simulink model "newest_singleprop"  (R2026b)
settings: Solver=VariableStepAuto  StopTime=60
values from neighbouring files (symbols this model uses):
  data_CP = static_data(:, 5)    [data_manipulation.m]    (also in initialize_propulsion.m)
  data_CT = static_data(:, 4)    [data_manipulation.m]    (also in initialize_propulsion.m)
  g = 9.81    [initialize_propulsion.m]    (also in run_comparisons.mat)
  prop_d = .0254 * prop_inches    (= 0.4318)    [initialize_propulsion.m]    (also in run_comparisons.mat)
  rho_reference = 1.212    [analyze_prop_db.m]    (also in data_manipulation.m; initialize_propulsion.m)
  rho_sim = rho_reference    (= 1.212)    [data_manipulation.m]    (also in initialize_propulsion.m)
libraries: fl_lib x29, nesl_utility x16, sdl_lib x1, batteryecm_lib x1, ee_lib x1
settings Model: Creator=123na  LastModifiedBy=brielle
settings DataIOCC: InspectSignalLogs=on
settings OptimizationCC: BlockReduction=off  BufferReuse=off  DefaultParameterBehavior=Inlined
settings SimscapeCC: SimscapeUseEnergyAccounting=off

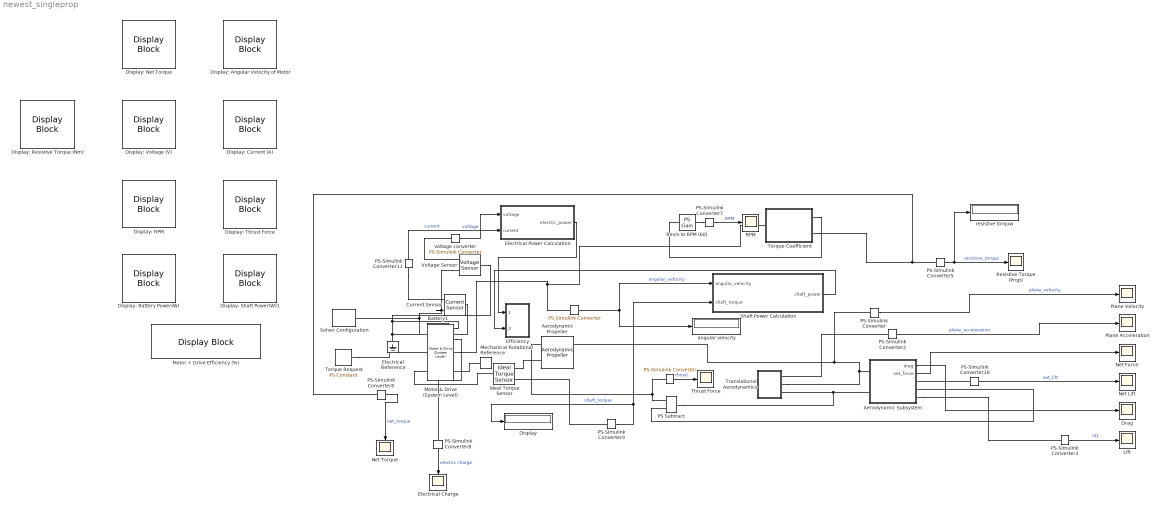
== system newest_singleprop ==
  " " : nesl_utility/PS-Simulink Converter  PhysicalDomain=network_engine_domain  SubClassName=ps_output  LeftPortType=input  RightPortType=output  PseudoPeriodic=off  Frequencies=[]  VectorFormat=inherit  Unit=N  AffineConversion=off
  "  " : nesl_utility/PS-Simulink Converter  PhysicalDomain=network_engine_domain  SubClassName=ps_output  LeftPortType=input  RightPortType=output  PseudoPeriodic=off  Frequencies=[]  VectorFormat=inherit  Unit=inherit  AffineConversion=off
  " Rev/s to RPM (60)" : fl_lib/Physical Signals/Functions/PS Gain  gain=60
  Aerodynamic Propeller : sdl_lib/Engines & Motors/Aerodynamic Propeller  parameterization=sdl.enum.AerodynamicPropellerParameterization.Constant  enable_collective_pitch_control=false  enable_transverse_flow=false  direction=sdl.enum.PropellerDirection.Positive  root_pitch=0 deg  D=prop_d m  kt_const=data_CT(4)  kp_const=data_CP(4)  kt_poly_fixed=[.002, .0006, -.0509, .0617]  kp_poly_fixed=[-.0752, .0577, -.0622, .16]  pitch_angle_TLU=[-15, 15, 25, 35, 45] deg  kt_poly_TLU=[.0002, -.00041, -.036, .03; .00026, -.00056, -.048, .04; .002, .00063, -.051, .062; .0014, -.0016, -.048, .087; .00087, -.0036, -.041, .12]  kp_poly_TLU=[-.1, .031, .0055, .088; -.081, -.025, .0044, .07; -.075, .058, -.062, .16; -.052, .065, -.08, .3; -.031, .057, -.069, .4]  J_TLU=[.01, .3, .625, 1.55, 2, 2.6]  kt_TLU_1D=[.0614, .0473, .0318, -.0127, -.0343, -.063]  kp_TLU_1D=[.1496, .1314, .116, -.0521, -.1503, -.2813]  kt_TLU_2D=[.00019, .013, .0048, -.017, -.03, -.045; .00039, .025, .0096, -.037, -.06, -.09; .00061, .047, .032, -.013, -.034, -.063; .00086, .072, .057, .014, -.0076, -.036; .12, .104, .09, .049, .029, .0019]  kp_TLU_2D=[.029, .029, .016, .06, .009, -.16; .059, .054, .031, -.12, -.19, -.29; .15, .13, .12, -.052, -.15, -.28; .26, .24, .22, .097, -.04, -.25; .39, .39, .38, .32, .24, .062]  beta_TLU=linspace(0, 360, 10) deg  Ct_TLU_1D=0.035 * sind(linspace(0, 360, 10) - 200)  Cq_TLU_1D=0.010 * sind(linspace(0, 360, 10) - 200)  Ct_TLU_2D=[0.01 * sind(linspace(0, 360, 10) - 200); 0.020 * sind(linspace(0, 360, 10) - 200); 0.035 * sind(linspace(0, 360, 10) - 200); 0.04 * sind(linspace(0, 360, 10) - 200); 0.06 * sind(linspace(0, 360, 10) - 200)]  Cq_TLU_2D=[0.0005 * sind(linspace(0, 360, 10) - 200); 0.0015 * sind(linspace(0, 360, 10) - 200); 0.0025 * sind(linspace(0, 360, 10) - 200); 0.0035 * sind(linspace(0, 360, 10) - 200); 0.0045 * sind(linspace(0, 360, 10) - 200)]  n_blades=2  radial_TLU=[.1, .12, .2, .4, .6, .8, 1]  twist_TLU=[30, 35, 50, 30, 20, 15, 10] deg  chord_TLU=[.0676, .0666, .0824, .1025, .0885, .0598, .0133]  alpha_TLU=-180 : 10 : 180 deg  Cl_TLU=[.1326, .1326, .1274, .1274, .1274, .1274, .1274; .3626, .3626, .5002, .5002, .5002, .5002, .5002; .5528, .5528, .8007, .8007, .8007, .8007, .8007; .7256, .7256, 1.0125, 1.0125, 1.0125, 1.0125, 1.0125; .8016, .8016, 1.1556, 1.1556, 1.1556, 1.1556, 1.1556; .7873, .7873, 1.1604, 1.1604, 1.1604, 1.1604, 1.1604; .7031, .7031, 1.0493, 1.0493, 1.0493, 1.0493, 1.0493; .5423, .5423, .7973, .7973, .7973, .7973, .7973; .3537, .3537, .4332, .4332, .4332, .4332, .4332; .1155, .1155, -.0376, -.0376, -.0376, -.0376, -.0376; -.1045, -.1045, -.4096, -.4096, -.4096, -.4096, -.4096; -.2999, -.2999, -.672, -.672, -.672, -.672, -.672; -.4401, -.4401, -.9343, -.9343, -.9343, -.9343, -.9343; -.5186, -.5186, -1.0477, -1.0477, -1.0477, -1.0477, -1.0477; -.5303, -.5303, -1.0387, -1.0387, -1.0387, -1.0387, -1.0387; -.5073, -.5073, -.9565, -.9565, -.9565, -.9565, -.9565; -.442, -.442, -.7713, -.7713, -.7713, -.7713, -.7713; -.2658, -.2658, -.4832, -.4832, -.4832, -.4832, -.4832; .4109, .4109, .3629, .3629, .3629, .3629, .3629; 1.1635, 1.1635, 1.3779, 1.3779, 1.3779, 1.3779, 1.3779; 1.2412, 1.2412, 1.4033, 1.4033, 1.4033, 1.4033, 1.4033; .7434, .7434, 1.3453, 1.3453, 1.3453, 1.3453, 1.3453; .7908, .7908, 1.2862, 1.2862, 1.2862, 1.2862, 1.2862; .7525, .7525, 1.1562, 1.1562, 1.1562, 1.1562, 1.1562; .6722, .6722, .9487, .9487, .9487, .9487, .9487; .5324, .5324, .7047, .7047, .7047, .7047, .7047; .3365, .3365, .382, .382, .382, .382, .382; .0529, .0529, -.0229, -.0229, -.0229, -.0229, -.0229; -.2728, -.2728, -.316, -.316, -.316, -.316, -.316; -.4135, -.4135, -.6195, -.6195, -.6195, -.6195, -.6195; -.5087, -.5087, -.7847, -.7847, -.7847, -.7847, -.7847; -.5342, -.5342, -.8419, -.8419, -.8419, -.8419, -.8419; -.5166, -.5166, -.7658, -.7658, -.7658, -.7658, -.7658; -.4321, -.4321, -.5707, -.5707, -.5707, -.5707, -.5707; -.2864, -.2864, -.3098, -.3098, -.3098, -.3098, -.3098; -.1073, -.1073, -.0893, -.0893, -.0893, -.0893, -.0893; .1326, .1326, .1274, .1274, .1274, .1274, .1274]  Cd_TLU=[.0055, .0055, .3904, .3904, .3904, .3904, .3904; .0774, .0774, .449, .449, .449, .449, .449; .2412, .2412, .5915, .5915, .5915, .5915, .5915; .4342, .4342, .8307, .8307, .8307, .8307, .8307; .679, .679, 1.0909, 1.0909, 1.0909, 1.0909, 1.0909; .9003, .9003, 1.3868, 1.3868, 1.3868, 1.3868, 1.3868; 1.0825, 1.0825, 1.6565, 1.6565, 1.6565, 1.6565, 1.6565; 1.2281, 1.2281, 1.875, 1.875, 1.875, 1.875, 1.875; 1.3205, 1.3205, 2.017, 2.017, 2.017, 2.017, 2.017; 1.3234, 1.3234, 2.0407, 2.0407, 2.0407, 2.0407, 2.0407; 1.2391, 1.2391, 1.9513, 1.9513, 1.9513, 1.9513, 1.9513; 1.0963, 1.0963, 1.7643, 1.7643, 1.7643, 1.7643, 1.7643; .8978, .8978, 1.5048, 1.5048, 1.5048, 1.5048, 1.5048; .6525, .6525, 1.2281, 1.2281, 1.2281, 1.2281, 1.2281; .4203, .4203, .838, .838, .838, .838, .838; .2428, .2428, .5434, .5434, .5434, .5434, .5434; .0951, .0951, .2517, .2517, .2517, .2517, .2517; .0292, .0292, .0698, .0698, .0698, .0698, .0698; .0148, .0148, .0267, .0267, .0267, .0267, .0267; .0808, .0808, .0509, .0509, .0509, .0509, .0509; .2429, .2429, .1561, .1561, .1561, .1561, .1561; .5019, .5019, .3927, .3927, .3927, .3927, .3927; .7217, .7217, .7438, .7438, .7438, .7438, .7438; .9336, .9336, 1.1277, 1.1277, 1.1277, 1.1277, 1.1277; 1.0984, 1.0984, 1.4838, 1.4838, 1.4838, 1.4838, 1.4838; 1.2274, 1.2274, 1.7877, 1.7877, 1.7877, 1.7877, 1.7877; 1.3016, 1.3016, 1.9779, 1.9779, 1.9779, 1.9779, 1.9779; 1.3305, 1.3305, 2.0516, 2.0516, 2.0516, 2.0516, 2.0516; 1.2889, 1.2889, 1.9974, 1.9974, 1.9974, 1.9974, 1.9974; 1.1677, 1.1677, 1.8463, 1.8463, 1.8463, 1.8463, 1.8463; 1.0076, 1.0076, 1.5699, 1.5699, 1.5699, 1.5699, 1.5699; .8068, .8068, 1.2596, 1.2596, 1.2596, 1.2596, 1.2596; .5688, .5688, .9493, .9493, .9493, .9493, .9493; .3604, .3604, .6154, .6154, .6154, .6154, .6154; .1802, .1802, .5015, .5015, .5015, .5015, .5015; .0699, .0699, .4265, .4265, .4265, .4265, .4265; .0055, .0055, .3904, .3904, .3904, .3904, .3904]  interp_method=simscape.enum.interpolation.linear  extrap_method=simscape.enum.extrapolation.linear  n_blade_discretization=10  n_azimuthal_discretization=10  density_spec=foundation.enum.constant_variable.constant  rho=rho_reference kg/m^3  rotational_ports=sdl.enum.ConnectionType.Conserving  translational_ports=sdl.enum.ConnectionType.PS  model_inertia=true  propeller_inertia=0.00001 kg*m^2  propeller_mass=10 kg  efficiency_sensor=false  n_thr=0.001 Hz  k_thr=0.001  P_thr=0.01 W  operation_check=simscape.enum.assert.action.warn  expose_port_C=false  w_specify=on  w_priority=High  w=0 rad/s  w_nominal_specify=off  w_nominal_value=1  w_nominal_unit=rad/s  Q_specify=off  Q_priority=None  Q=0 N*m  Q_nominal_specify=off  Q_nominal_value=1  Q_nominal_unit=N*m  v_specify=off  v_priority=None  v=0 m/s  v_nominal_specify=off  v_nominal_value=1  v_nominal_unit=m/s  thrust_specify=off  thrust_priority=None  thrust=0 N  thrust_nominal_specify=off  thrust_nominal_value=1  thrust_nominal_unit=N
  Aerodynamic Subsystem : Subsystem
  Battery1 : batteryecm_lib/Battery  Vnom=22.2 V  prm_dir=simscape.enum.battery.prm_dir.disabled  R1_dis=2 Ohm  R1_ch=2 Ohm  R1=15 mOhm  prm_AH=simscape.enum.battery.prm_AH.finite  AH=4 A*hr  V1=21.3 V  AH1=0.48 Ah  prm_R2=simscape.enum.battery.prm_R2.disabled  R2=2000 Ohm  Tmeas=298.15 K  charge_measurement_port=simscape.enum.battery.enable.yes  prm_dyn=simscape.enum.battery.prm_dyn.off  Rp1=0.005 Ohm  tau1=30 s  Rp2=0.005 Ohm  tau2=30 s  Rp3=0.005 Ohm  tau3=30 s  Rp4=0.005 Ohm  tau4=30 s  Rp5=0.005 Ohm  tau5=30 s  prm_fade=simscape.enum.battery.prm_fade.disabled  N_fade=100  AH_fade=45 A*hr  R1_fade=2.02 Ohm  R1_ch_fade=2.02 Ohm  V1_fade=10.35 V  prm_age=simscape.enum.battery.prm_age.disabled  prm_age_OCV=simscape.enum.battery.prm_age_OCV.OCV  OCV_age=0.9  SOC_age=60  Tmeas_age=298.15 K  delta_time_age_vec=[0] d  temperature_age_vec=[273] K  OCV_scaling_age=2.2134e6  OCV_offset_age=1.632e6  temp_exp_age=0.515833569 V  t_exp_age=0.75  Vnom_T2=12 V  R1_T2=2.2 Ohm  R1_T2_dis=2.2 Ohm  R1_T2_ch=2.2 Ohm  V1_T2=11.4 V  R2_T2=2200 Ohm  Rp1_T2=0.005 Ohm  tau1_T2=30 s  Rp2_T2=0.005 Ohm  tau2_T2=30 s  Rp3_T2=0.005 Ohm  tau3_T2=30 s  Rp4_T2=0.005 Ohm  tau4_T2=30 s  Rp5_T2=0.005 Ohm  tau5_T2=30 s  Tmeas2=273.15 K  thermal_port=simscape.enum.thermaleffects.omit  thermal_mass=30000 J/K  i_specify=off  i_priority=None  i=0 A  i_nominal_specify=off  i_nominal_value=1  i_nominal_unit=A  v_specify=off  v_priority=None  v=0 V  v_nominal_specify=off  v_nominal_value=1  v_nominal_unit=V  charge_specify=off  charge_priority=High  charge=50 A*hr  charge_nominal_specify=off  charge_nominal_value=1  charge_nominal_unit=A*hr  num_cycles_specify=off  num_cycles_priority=High  num_cycles=0  num_cycles_nominal_specify=off  num_cycles_nominal_value=1  num_cycles_nominal_unit=1  temperature_specify=off  temperature_priority=High  temperature=298.15 K  temperature_nominal_specify=off  temperature_nominal_value=1  temperature_nominal_unit=K
      settings: LibrarySourceBlock=batt_lib/Cells/Battery
  Current Sensor : fl_lib/Electrical/Electrical Sensors/Current Sensor
  Display : Display
  Display: Angular Velocity of Motor : DisplayBlock  LabelPosition=Hide  Transparency=1  GridColor=[0.502, 0.502, 0.502]
  Display: Battery Power(W) : DisplayBlock  LabelPosition=Hide  Format=Integer  Transparency=1  GridColor=[0.0, 0.0, 1.0]
  Display: Current (A) : DisplayBlock  LabelPosition=Hide  Transparency=1  GridColor=[0.502, 0.502, 0.502]
  Display: Net Torque : DisplayBlock  LabelPosition=Hide  Transparency=1  GridColor=[0.502, 0.502, 0.502]
  Display: RPM : DisplayBlock  LabelPosition=Hide  Format=Integer  Transparency=1  GridColor=[0.0, 0.0, 1.0]
  Display: Resistive Torque (Nm) : DisplayBlock  LabelPosition=Hide  Transparency=1  GridColor=[0.502, 0.502, 0.502]
  Display: Shaft Power(W)1 : DisplayBlock  LabelPosition=Hide  Transparency=1  GridColor=[0.0, 0.0, 1.0]
  Display: Thrust Force : DisplayBlock  LabelPosition=Hide  Transparency=1  GridColor=[0.502, 0.502, 0.502]
  Display: Voltage (V) : DisplayBlock  LabelPosition=Hide  Transparency=1  GridColor=[0.502, 0.502, 0.502]
  Drag : Scope
      settings: ActiveDisplayYMinimum=-14.344967530290399  ActiveDisplayYMaximum=129.10470777261361  DataLoggingVariableName=ScopeData8
  Efficiency : Subsystem
  Electrical Charge : Scope
      settings: ActiveDisplayYMinimum=160492.22040625822  ActiveDisplayYMaximum=182167.5310659713  DataLoggingVariableName=ScopeData10
  Electrical Power Calculation : Subsystem
  Electrical Reference : fl_lib/Electrical/Electrical Elements/Electrical Reference
  Ideal Torque Sensor : fl_lib/Mechanical/Mechanical Sensors/Ideal Torque Sensor
  Lift : Scope
      settings: ActiveDisplayYMinimum=-49.526573340247545  ActiveDisplayYMaximum=445.73916006222805  DataLoggingVariableName=ScopeData7
  Mechanical Rotational Reference : fl_lib/Mechanical/Rotational Elements/Mechanical Rotational Reference
  Motor & Drive (System Level) : ee_lib/Electromechanical/Motor & Drive (System Level)  torque_speed_param=ee.enum.electromech.envelope.torque_power  overtorque_param=ee.enum.electromech.overtorque.no  T_t=[.09, .08, .07, 0] N*m  T_t_intermittent=[.36, .32, .28, 0] N*m  T_t_2D=[.09, .09, .09; .08, .08, .08; .07, .07, .07; 0, 0, 0] N*m  T_t_intermittent_2D=[.36, .36, .36; .32, .32, .32; .28, .28, .28; 0, 0, 0] N*m  w_t=[0, 3750, 7500, 8000] rpm  vdc_t=[6, 12, 24] V  torque_max=5.5 N*m  power_max=900 W  torque_max_intermittent=0.4 N*m  power_max_intermittent=120 W  time_overtorque=30 s  time_recover=60 s  Tc=0.02 s  EnableSwitch=false  losses_param=1  eff=88  w_eff=6000 rpm  T_eff=4 N*m  Piron=0 W  Pbase=0 W  w_eff_vec=[-8000, -4000, 0, 4000, 8000] rpm  T_eff_vec=[0, .03, .06, .09] N*m  v_eff_vec=[100, 250, 400] V  losses_mat=[1.49, 1.67, 2.21, 3.1; .42, .69, 1.14, 2.03; .06, .24, .78, 1.68; .42, .69, 1.14, 2.03; 1.49, 1.67, 2.21, 3.1] W  efficiency_mat=[95, 95, 95, 95; 95, 95, 95, 95; 95, 95, 95, 95; 95, 95, 95, 95; 95, 95, 95, 95]  losses_mat_3D=ones(5, 4, 3) W  efficiency_mat_3D=95 * ones(5, 4, 3)  Res=0.016 Ohm  J=5e-6 kg*m^2  lam=1e-5 N*m*s/rad  speed0=0 rpm  faulted_specify=off  faulted_priority=None  faulted=0  faulted_nominal_specify=off  faulted_nominal_value=1  faulted_nominal_unit=1  isSwitchedOff_specify=off  isSwitchedOff_priority=None  isSwitchedOff=0  isSwitchedOff_nominal_specify=off  isSwitchedOff_nominal_value=1  isSwitchedOff_nominal_unit=1  torqueLimitContinuous_specify=off  torqueLimitContinuous_priority=None  torqueLimitContinuous=0 N*m  torqueLimitContinuous_nominal_specify=off  torqueLimitContinuous_nominal_value=1  torqueLimitContinuous_nominal_unit=N*m  TabulateLossesForMultipleTemperatures=false  alpha=3.93e-3 1/K  Tmeas=25 degC  TmeasVec=[25, 75, 125] degC  Tmeas2=125 degC  losses_mat_T2=[1.49, 1.74, 2.49, 3.74; .42, .67, 1.42, 2.67; .06, .31, 1.06, 2.31; .42, .67, 1.42, 2.67; 1.49, 1.74, 2.49, 3.74] W  efficiency_mat_T2=[95, 95, 95, 95; 95, 95, 95, 95; 95, 95, 95, 95; 95, 95, 95, 95; 95, 95, 95, 95]  losses_mat_3D_T2=ones(5, 4, 3) W  efficiency_mat_3D_T2=95 * ones(5, 4, 3)  lossesMatMultipleTemperatures=ones(5, 4, 3) W  efficiencyMatMultipleTemperatures=95 * ones(5, 4, 3)  lossesMat4DMultipleTemperatures=ones(5, 4, 3, 3) W  efficiencyMat4DMultipleTemperatures=95 * ones(5, 4, 3, 3)  thermal_mass=100 J/K  initial_temperature=25 degC
  Motor + Drive Efficiency (%) : DisplayBlock  LabelPosition=Hide  Transparency=1  GridColor=[0.0, 0.0, 1.0]
  Net Force : Scope
      settings: ActiveDisplayYMinimum=-4.5427625845531994  ActiveDisplayYMaximum=40.884863260978804  DataLoggingVariableName=ScopeData5
  Net Lift : Scope
      settings: ActiveDisplayYMinimum=-156.32019566352511  ActiveDisplayYMaximum=338.9455409717259  DataLoggingVariableName=ScopeData12
  Net Torque : Scope
      settings: ActiveDisplayYMinimum=2.5365925575733379  ActiveDisplayYMaximum=5.2737119380474073  DataLoggingVariableName=ScopeData4
  PS Subtract : fl_lib/Physical Signals/Functions/PS Subtract
  PS-Simulink Converter{,2..3,5..10} (9 alike) : nesl_utility/PS-Simulink Converter  PhysicalDomain=network_engine_domain  SubClassName=ps_output  LeftPortType=input  RightPortType=output  PseudoPeriodic=off  Frequencies=[]  VectorFormat=inherit  Unit=inherit  AffineConversion=off
  PS-Simulink Converter11 : nesl_utility/PS-Simulink Converter  PhysicalDomain=network_engine_domain  SubClassName=ps_output  LeftPortType=input  RightPortType=output  PseudoPeriodic=off  Frequencies=[]  VectorFormat=inherit  Unit=A  AffineConversion=off
  Plane Acceleration : Scope
      settings: ActiveDisplayYMinimum=-0.565213030160767  ActiveDisplayYMaximum=5.0869172714469038
  Plane Velocity : Scope
      settings: ActiveDisplayYMinimum=-4.7776171506476794  ActiveDisplayYMaximum=42.998554355829121  DataLoggingVariableName=ScopeData6
  RPM : Scope
      settings: ActiveDisplayYMinimum=-379.69821594020021  ActiveDisplayYMaximum=3417.2839434618027  DataLoggingVariableName=ScopeData9
  Resistive Torque (Prop) : Scope
      settings: ActiveDisplayYMinimum=-0.15553318378531714  ActiveDisplayYMaximum=1.3997986540678544  DataLoggingVariableName=ScopeData3
  Shaft Power Calculation : Subsystem
  Solver Configuration : nesl_utility/Solver Configuration  PhysicalDomain=network_engine_domain  SubClassName=solver  LeftPortType=input  RightPortType=generic  Tones=[]  Harmonics=[]  SimulateNoise=off  Profile=off  UseLocalSampling=off  EnableSwitchedLinearOptims=on  FrequencyDomain=off  UseCCode=off  RelTol=0.001  AbsTol=0.001  MinStep=1e-09  ToWorkspace=off  RevertToSquareIcSolve=off  NumHomotopyIterations=100  PhasorMode=off  PhasorModeNumHarmonics=1  ConsistencySolver=NEWTON_XTOL_AFTER_FTOL  CanonicalOrdering=UNORDERED  OptimizeIntermediates=UNOPTIMIZED  MulticoreSolverChoice=BACKWARD_EULER  IndexReductionMethod=DerivativeReplacement  DoDC=off  ResidualTolerance=1e-09  ConsistencyTolSource=GLOBAL  ConsistencyAbsTol=0.001  ConsistencyRelTol=0.001  ConsistencyTolFactor=0.001  UseLocalSolver=off  LocalSolverChoice=NE_BACKWARD_EULER_ADVANCER  ResolveIndetEquations=on  FunctionEvalNumThread=1  LocalSolverSampleTime=0.001  DoFixedCost=off  MaxNonlinIter=3  MaxModeIter=2  ComputeImpulses=off  ImpulseIterations=2  LinearAlgebra=auto  LinearAlgebraNumThread=0  EquationFormulation=NE_TIME_EF  DelaysMemoryBudget=1024  AutomaticFiltering=on  FilteringTimeConstant=0.001  PartitionStorageMethod=AS_NEEDED  PartitionMemoryBudget=1024  PartitionMethod=BALANCED  MultibodyUseLocalSolver=off  MultibodyLocalSolverChoice=ODE1  MultibodyLocalSolverSampleTime=0.001
  "Thrust Force " : Scope
      settings: ActiveDisplayYMinimum=-7.0175807682346578  ActiveDisplayYMaximum=63.158226914111935
  Torque Coefficient : Subsystem
  Torque Request : fl_lib/Physical Signals/Sources/PS Constant  constant=2.15 N*m
  Translational Aerodynamics : Subsystem
  Voltage Sensor : fl_lib/Electrical/Electrical Sensors/Voltage Sensor
  angular velocity : Display
  resistive torquw : Display
  voltage converter : nesl_utility/PS-Simulink Converter  PhysicalDomain=network_engine_domain  SubClassName=ps_output  LeftPortType=input  RightPortType=output  PseudoPeriodic=off  Frequencies=[]  VectorFormat=inherit  Unit=inherit  AffineConversion=off
  wires:
  " "/1 -> "Thrust Force "/1  "thrust"
  PS-Simulink Converter/1 -> Plane Velocity/1  "plane_velocity"
  PS-Simulink Converter2/1 -> Plane Acceleration/1  "plane_acceleration"
  PS-Simulink Converter3/1 -> Lift/1  "lift"
  PS-Simulink Converter6/1 -> Net Torque/1  "net_torque"
  PS-Simulink Converter5/1 -> resistive torquw/1, Resistive Torque (Prop)/1  "resistive_torque"
  PS-Simulink Converter7/1 -> RPM/1  "RPM"
  PS-Simulink Converter8/1 -> Electrical Charge/1  "electric charge"
  PS-Simulink Converter10/1 -> Net Lift/1  "net_lift"
  "  "/1 -> Shaft Power Calculation/1(angular_velocity), angular velocity/1  "angular_velocity"
  voltage converter/1 -> Electrical Power Calculation/1(voltage)  "voltage"
  PS-Simulink Converter11/1 -> Electrical Power Calculation/2(current)  "current"
  Electrical Power Calculation/1(electric_power) -> Efficiency/1(electrical power)
  Aerodynamic Subsystem/1(drag) -> Drag/1
  Aerodynamic Subsystem/2(net_force) -> Net Force/1
  PS-Simulink Converter9/1 -> Display/1, Shaft Power Calculation/2(shaft_torque)  "shaft_torque"
  Shaft Power Calculation/1(shaft_power) -> Efficiency/2(shaft power)
  connections:
  Motor & Drive (System Level)/LConn1 -- Voltage Sensor/LConn1 -- Battery1/LConn1 -- Electrical Reference/LConn1
  Voltage Sensor/RConn2 -- Current Sensor/RConn2 -- Battery1/RConn1 -- Solver Configuration/RConn1
  Motor & Drive (System Level)/RConn3 -- Mechanical Rotational Reference/LConn1
  Motor & Drive (System Level)/RConn2 -- Torque Coefficient/LConn1 -- "  "/LConn1
  " "/LConn1 -- Aerodynamic Propeller/LConn1 -- PS Subtract/LConn1
  Torque Request/RConn1 -- Motor & Drive (System Level)/LConn2
  Torque Coefficient/RConn2 -- PS-Simulink Converter6/LConn1 -- PS-Simulink Converter5/LConn1
  " Rev/s to RPM (60)"/RConn1 -- PS-Simulink Converter7/LConn1
  Battery1/LConn2 -- PS-Simulink Converter8/LConn1
  Voltage Sensor/RConn1 -- voltage converter/LConn1
  Motor & Drive (System Level)/RConn1 -- Current Sensor/LConn1
  PS-Simulink Converter11/LConn1 -- Current Sensor/RConn1
  PS-Simulink Converter9/LConn1 -- Ideal Torque Sensor/RConn2
  Ideal Torque Sensor/RConn1 -- Aerodynamic Propeller/LConn2
  Motor & Drive (System Level)/LConn3 -- Ideal Torque Sensor/LConn1
  Torque Coefficient/RConn1 -- " Rev/s to RPM (60)"/LConn1
  PS-Simulink Converter2/LConn1 -- Translational Aerodynamics/RConn1
  Translational Aerodynamics/RConn2 -- PS-Simulink Converter/LConn1 -- Aerodynamic Propeller/RConn1 -- Aerodynamic Subsystem/LConn1
  Translational Aerodynamics/RConn3 -- PS Subtract/RConn1 -- Aerodynamic Subsystem/LConn2
  PS-Simulink Converter10/LConn1 -- Aerodynamic Subsystem/RConn1
  PS Subtract/LConn2 -- Aerodynamic Subsystem/RConn2
  Aerodynamic Subsystem/RConn3 -- PS-Simulink Converter3/LConn1

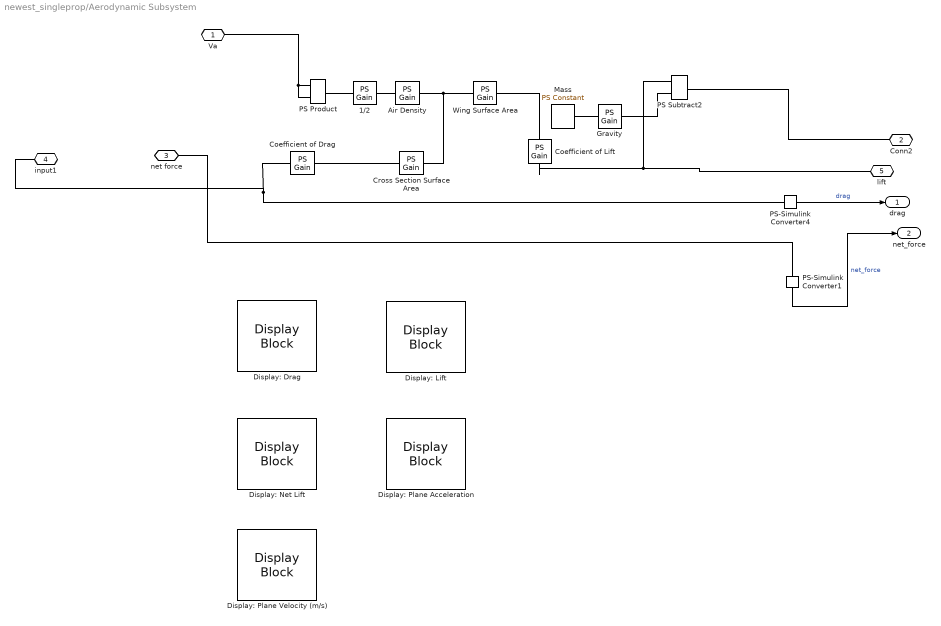
== system newest_singleprop/Aerodynamic Subsystem ==
  1/2 : fl_lib/Physical Signals/Functions/PS Gain  gain=.5
  Air Density : fl_lib/Physical Signals/Functions/PS Gain  gain=rho_sim kg/m^3
  Coefficient of Drag : fl_lib/Physical Signals/Functions/PS Gain  gain=0.06
  Coefficient of Lift : fl_lib/Physical Signals/Functions/PS Gain  gain=.58
  Cross Section Surface Area : fl_lib/Physical Signals/Functions/PS Gain  gain=1.0448384 m^2
  Display: Drag : DisplayBlock  LabelPosition=Hide  Transparency=1  GridColor=[0.502, 0.502, 0.502]
  Display: Lift : DisplayBlock  LabelPosition=Hide  Transparency=1  GridColor=[0.502, 0.502, 0.502]
  Display: Net Lift : DisplayBlock  LabelPosition=Hide  Transparency=1  GridColor=[0.502, 0.502, 0.502]
  Display: Plane Acceleration : DisplayBlock  LabelPosition=Hide  Transparency=1  GridColor=[0.502, 0.502, 0.502]
  Display: Plane Velocity (m/s) : DisplayBlock  LabelPosition=Hide  Transparency=1  GridColor=[0.502, 0.502, 0.502]
  Gravity : fl_lib/Physical Signals/Functions/PS Gain  gain=g m/(s^2)
  Mass : fl_lib/Physical Signals/Sources/PS Constant  constant=mass kg
  PS Product : fl_lib/Physical Signals/Functions/PS Product
  PS Subtract2 : fl_lib/Physical Signals/Functions/PS Subtract
  PS-Simulink Converter1 : nesl_utility/PS-Simulink Converter  PhysicalDomain=network_engine_domain  SubClassName=ps_output  LeftPortType=input  RightPortType=output  PseudoPeriodic=off  Frequencies=[]  VectorFormat=inherit  Unit=inherit  AffineConversion=off
  PS-Simulink Converter4 : nesl_utility/PS-Simulink Converter  PhysicalDomain=network_engine_domain  SubClassName=ps_output  LeftPortType=input  RightPortType=output  PseudoPeriodic=off  Frequencies=[]  VectorFormat=inherit  Unit=inherit  AffineConversion=off
  Wing Surface Area : fl_lib/Physical Signals/Functions/PS Gain  gain=0.87 m^2
  Va : PMIOPort  Side=Left
  Conn2 : PMIOPort  Port=2  Side=Right
  net force : PMIOPort  Port=3  Side=Left
  input1 : PMIOPort  Port=4  Side=Right
  lift : PMIOPort  Port=5  Side=Right
  drag : Outport
  net_force : Outport  Port=2
  wires:
  PS-Simulink Converter1/1 -> net_force/1  "net_force"
  PS-Simulink Converter4/1 -> drag/1  "drag"
  connections:
  Conn2/RConn1 -- PS Subtract2/RConn1
  Coefficient of Lift/LConn1 -- Wing Surface Area/RConn1
  Wing Surface Area/LConn1 -- Cross Section Surface Area/LConn1 -- Air Density/RConn1
  PS Product/RConn1 -- 1/2/LConn1
  Air Density/LConn1 -- 1/2/RConn1
  Gravity/RConn1 -- PS Subtract2/LConn2
  Gravity/LConn1 -- Mass/RConn1
  PS Product/LConn1 -- PS Product/LConn2 -- Va/RConn1
  PS-Simulink Converter1/LConn1 -- net force/RConn1
  Cross Section Surface Area/RConn1 -- Coefficient of Drag/LConn1
  Coefficient of Drag/RConn1 -- input1/RConn1 -- PS-Simulink Converter4/LConn1
  Coefficient of Lift/RConn1 -- PS Subtract2/LConn1 -- lift/RConn1

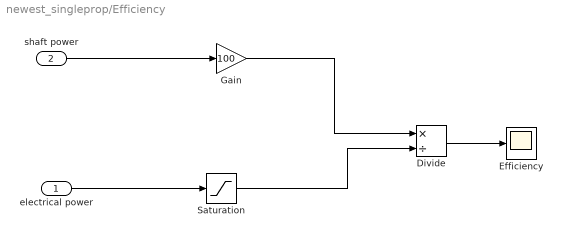
== system newest_singleprop/Efficiency ==
  electrical power : Inport
  shaft power : Inport  Port=2
  Divide : Product  Inputs=*/
  Efficiency : Scope
      settings: ActiveDisplayYMinimum=-54.765164223208942  ActiveDisplayYMaximum=492.8864780088806  DataLoggingVariableName=ScopeData14
  Gain : Gain  Gain=100
  Saturation : Saturate  UpperLimit=inf  LowerLimit=.0001
  wires:
  shaft power/1 -> Gain/1
  electrical power/1 -> Saturation/1
  Divide/1 -> Efficiency/1
  Saturation/1 -> Divide/2
  Gain/1 -> Divide/1

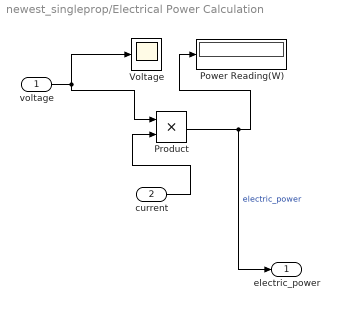
== system newest_singleprop/Electrical Power Calculation ==
  voltage : Inport
  current : Inport  Port=2
  Power Reading(W) : Display
  Product : Product
  Voltage : Scope
      settings: ActiveDisplayYMinimum=21.504198233190788  ActiveDisplayYMaximum=22.408763563943079  DataLoggingVariableName=ScopeData11
  electric_power : Outport
  wires:
  current/1 -> Product/2
  Product/1 -> electric_power/1, Power Reading(W)/1  "electric_power"
  voltage/1 -> Product/1, Voltage/1

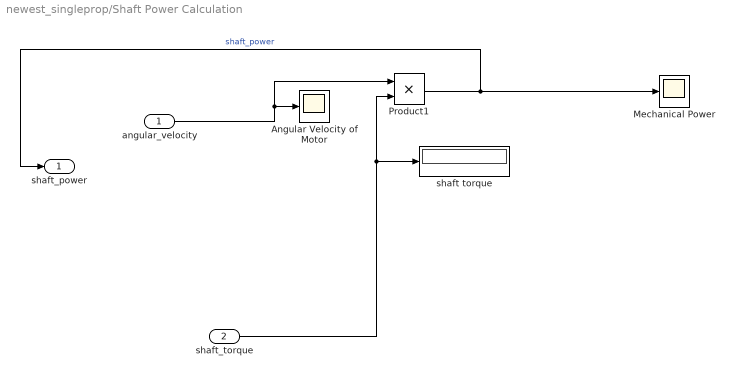
== system newest_singleprop/Shaft Power Calculation ==
  angular_velocity : Inport
  shaft_torque : Inport  Port=2
  Angular Velocity of Motor : Scope
      settings: ActiveDisplayYMinimum=-54.765164223208942  ActiveDisplayYMaximum=492.8864780088806  DataLoggingVariableName=ScopeData2
  Mechanical Power : Scope
      settings: ActiveDisplayYMinimum=-112.00431950769796  ActiveDisplayYMaximum=1008.0388755692819  DataLoggingVariableName=ScopeData13
  Product1 : Product
  shaft torque : Display
  shaft_power : Outport
  wires:
  shaft_torque/1 -> shaft torque/1, Product1/2
  angular_velocity/1 -> Product1/1, Angular Velocity of Motor/1
  Product1/1 -> shaft_power/1, Mechanical Power/1  "shaft_power"

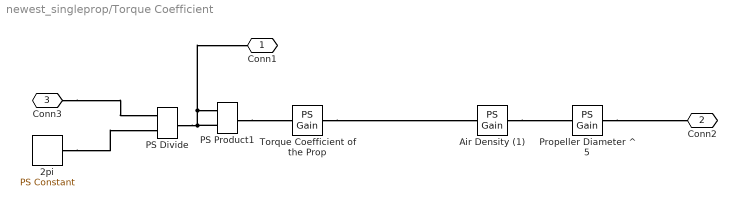
== system newest_singleprop/Torque Coefficient ==
  2pi : fl_lib/Physical Signals/Sources/PS Constant  constant=rad rad
  Air Density (1) : fl_lib/Physical Signals/Functions/PS Gain  gain=rho_reference kg/(m^3)
  PS Divide : fl_lib/Physical Signals/Functions/PS Divide
  PS Product1 : fl_lib/Physical Signals/Functions/PS Product
  Propeller Diameter ^ 5 : fl_lib/Physical Signals/Functions/PS Gain  gain=prop_d^5 m^5
  Torque Coefficient of the Prop : fl_lib/Physical Signals/Functions/PS Gain  gain=data_CP(4)/(2*pi)
  Conn1 : PMIOPort  Side=Right
  Conn2 : PMIOPort  Port=2  Side=Right
  Conn3 : PMIOPort  Port=3  Side=Left
  connections:
  Air Density (1)/RConn1 -- Propeller Diameter ^ 5/LConn1
  Torque Coefficient of the Prop/RConn1 -- Air Density (1)/LConn1
  Conn3/RConn1 -- PS Divide/LConn1
  PS Product1/RConn1 -- Torque Coefficient of the Prop/LConn1
  Propeller Diameter ^ 5/RConn1 -- Conn2/RConn1
  2pi/RConn1 -- PS Divide/LConn2
  PS Divide/RConn1 -- PS Product1/LConn2 -- Conn1/RConn1 -- PS Product1/LConn1

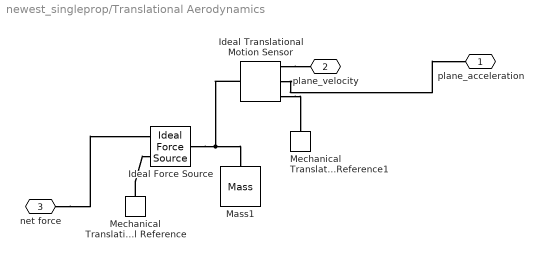
== system newest_singleprop/Translational Aerodynamics ==
  Ideal Force Source : fl_lib/Mechanical/Mechanical Sources/Ideal Force Source
  Ideal Translational Motion Sensor : fl_lib/Mechanical/Mechanical Sensors/Ideal Translational Motion Sensor  reference=foundation.enum.MeasurementReference.difference  acceleration_port=true  velocity_port=true  position_port=false  offset=0 m
  Mass1 : fl_lib/Mechanical/Translational Elements/Mass  mass=mass kg  num_ports=foundation.enum.numPorts2.one  v_specify=off  v_priority=High  v=0 m/s  v_nominal_specify=off  v_nominal_value=1  v_nominal_unit=m/s  f_specify=off  f_priority=None  f=0 N  f_nominal_specify=off  f_nominal_value=1  f_nominal_unit=N
  Mechanical Translational Reference : fl_lib/Mechanical/Translational Elements/Mechanical Translational Reference
  Mechanical Translational Reference1 : fl_lib/Mechanical/Translational Elements/Mechanical Translational Reference
  plane_acceleration : PMIOPort  Side=Right
  plane_velocity : PMIOPort  Port=2  Side=Right
  net force : PMIOPort  Port=3  Side=Right
  connections:
  net force/RConn1 -- Ideal Force Source/RConn1
  Ideal Translational Motion Sensor/RConn2 -- plane_acceleration/RConn1
  Mechanical Translational Reference/LConn1 -- Ideal Force Source/RConn2
  Ideal Translational Motion Sensor/RConn1 -- Mechanical Translational Reference1/LConn1
  Ideal Translational Motion Sensor/RConn3 -- plane_velocity/RConn1
  Ideal Force Source/LConn1 -- Ideal Translational Motion Sensor/LConn1 -- Mass1/LConn1
